simulink model "sgact"  (R2026b)
settings: Solver=FixedStepDiscrete  StopTime=inf  FixedStep=0.001
PreLoadFcn:
  | addpath(fullfile(fileparts(which('sgact')), 'matlab')); sgact_buses;
undefined symbols (not defined in the file or in its folder): sgact_sp_default
libraries: sgact_lib x4
settings Model: Creator=maccame  LastModifiedBy=maccame
settings SolverCC: ConcurrentTasks=on  PositivePriorityOrder=on
settings OptimizationCC: BlockReduction=off  DefaultParameterBehavior=Inlined  OptimizeBlockIOStorage=off
settings DebuggingCC: TasksWithSamePriorityMsg=none
settings HardwareCC: ProdHWDeviceType=Intel->x86-64 (Linux 64)  ProdLongLongMode=on
settings RTWCC: BuildConfiguration=Faster Runs  Description=Speedgoat Real-Time Target Machine  SystemTargetFile=speedgoat.tlc  TargetLang=C++  TemplateMakefile=slrealtime_default_tmf  Toolchain=Simulink Real-Time Toolchain
settings SimulinkRealTimeTargetCC: MATLABClassNameForMDSCustomization=Simulink.SoftwareTarget.GRTCustomization  TargetLangStandard=C++11 (ISO)

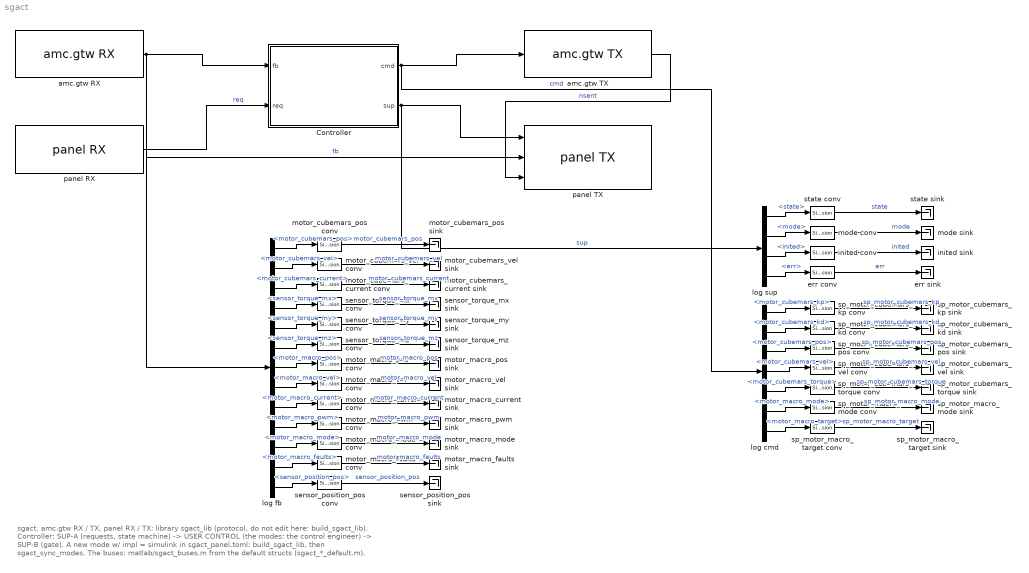
== system sgact ==
  note: sgact. amc.gtw RX / TX, panel RX / TX: library sgact_lib (protocol, do not edit here: build_sgact_lib).
      | Controller: SUP-A (requests, state machine) -> USER CONTROL (the modes: the control engineer) -> SUP-B (gate).
      | A new mode w/ impl = simulink in sgact_panel.toml: build_sgact_lib, then sgact_sync_modes.
      | The buses: matlab/sgact_buses.m from the default structs (sgact_*_default.m).
  Controller : Subsystem
  amc.gtw RX : sgact_lib/amc.gtw RX  SystemSampleTime=-1  VariantActivationTime=update diagram  EmptyChoice=off  PassThrough=off  PassThroughVariantControl=(default)  EmptyChoiceVariantControl=(default)  AllowFlexibleInterface=on  Latency=0  AutoFrameSizeCalculation=off
  amc.gtw TX : sgact_lib/amc.gtw TX  SystemSampleTime=-1  VariantActivationTime=update diagram  EmptyChoice=off  PassThrough=off  PassThroughVariantControl=(default)  EmptyChoiceVariantControl=(default)  AllowFlexibleInterface=on  Latency=0  AutoFrameSizeCalculation=off
  err conv : SignalConversion  OverrideOpt=off
  err sink : Terminator
  inited conv : SignalConversion  OverrideOpt=off
  inited sink : Terminator
  log cmd : BusSelector  OutputSignals=motor_cubemars_kp,motor_cubemars_kd,motor_cubemars_pos,motor_cubemars_vel,motor_cubemars_torque,motor_macro_mode,motor_macro_target
  log fb : BusSelector  OutputSignals=motor_cubemars_pos,motor_cubemars_vel,motor_cubemars_current,sensor_torque_mx,sensor_torque_my,sensor_torque_mz,motor_macro_pos,motor_macro_vel,motor_macro_current,motor_macro_pwm,motor_macro_mode,motor_macro_faults,sensor_position_pos
  log sup : BusSelector  OutputSignals=state,mode,inited,err
  mode conv : SignalConversion  OverrideOpt=off
  mode sink : Terminator
  motor_cubemars_current conv : SignalConversion  OverrideOpt=off
  motor_cubemars_current sink : Terminator
  motor_cubemars_pos conv : SignalConversion  OverrideOpt=off
  motor_cubemars_pos sink : Terminator
  motor_cubemars_vel conv : SignalConversion  OverrideOpt=off
  motor_cubemars_vel sink : Terminator
  motor_macro_current conv : SignalConversion  OverrideOpt=off
  motor_macro_current sink : Terminator
  motor_macro_faults conv : SignalConversion  OverrideOpt=off
  motor_macro_faults sink : Terminator
  motor_macro_mode conv : SignalConversion  OverrideOpt=off
  motor_macro_mode sink : Terminator
  motor_macro_pos conv : SignalConversion  OverrideOpt=off
  motor_macro_pos sink : Terminator
  motor_macro_pwm conv : SignalConversion  OverrideOpt=off
  motor_macro_pwm sink : Terminator
  motor_macro_vel conv : SignalConversion  OverrideOpt=off
  motor_macro_vel sink : Terminator
  panel RX : sgact_lib/panel RX  SystemSampleTime=-1  VariantActivationTime=update diagram  EmptyChoice=off  PassThrough=off  PassThroughVariantControl=(default)  EmptyChoiceVariantControl=(default)  AllowFlexibleInterface=on  Latency=0  AutoFrameSizeCalculation=off
  panel TX : sgact_lib/panel TX  SystemSampleTime=-1  VariantActivationTime=update diagram  EmptyChoice=off  PassThrough=off  PassThroughVariantControl=(default)  EmptyChoiceVariantControl=(default)  AllowFlexibleInterface=on  Latency=0  AutoFrameSizeCalculation=off
  sensor_position_pos conv : SignalConversion  OverrideOpt=off
  sensor_position_pos sink : Terminator
  sensor_torque_mx conv : SignalConversion  OverrideOpt=off
  sensor_torque_mx sink : Terminator
  sensor_torque_my conv : SignalConversion  OverrideOpt=off
  sensor_torque_my sink : Terminator
  sensor_torque_mz conv : SignalConversion  OverrideOpt=off
  sensor_torque_mz sink : Terminator
  sp_motor_cubemars_kd conv : SignalConversion  OverrideOpt=off
  sp_motor_cubemars_kd sink : Terminator
  sp_motor_cubemars_kp conv : SignalConversion  OverrideOpt=off
  sp_motor_cubemars_kp sink : Terminator
  sp_motor_cubemars_pos conv : SignalConversion  OverrideOpt=off
  sp_motor_cubemars_pos sink : Terminator
  sp_motor_cubemars_torque conv : SignalConversion  OverrideOpt=off
  sp_motor_cubemars_torque sink : Terminator
  sp_motor_cubemars_vel conv : SignalConversion  OverrideOpt=off
  sp_motor_cubemars_vel sink : Terminator
  sp_motor_macro_mode conv : SignalConversion  OverrideOpt=off
  sp_motor_macro_mode sink : Terminator
  sp_motor_macro_target conv : SignalConversion  OverrideOpt=off
  sp_motor_macro_target sink : Terminator
  state conv : SignalConversion  OverrideOpt=off
  state sink : Terminator
  wires:
  amc.gtw RX/1 -> Controller/1(fb), panel TX/2, log fb/1  "fb"
  panel RX/1 -> Controller/2(req)  "req"
  Controller/1(cmd) -> amc.gtw TX/1, log cmd/1  "cmd"
  Controller/2(sup) -> panel TX/1, log sup/1  "sup"
  amc.gtw TX/1 -> panel TX/3  "nsent"
  log sup/1 -> state conv/1  "<state>"
  state conv/1 -> state sink/1  "state"
  log sup/2 -> mode conv/1  "<mode>"
  mode conv/1 -> mode sink/1  "mode"
  log sup/3 -> inited conv/1  "<inited>"
  inited conv/1 -> inited sink/1  "inited"
  log sup/4 -> err conv/1  "<err>"
  err conv/1 -> err sink/1  "err"
  log cmd/1 -> sp_motor_cubemars_kp conv/1  "<motor_cubemars_kp>"
  sp_motor_cubemars_kp conv/1 -> sp_motor_cubemars_kp sink/1  "sp_motor_cubemars_kp"
  log cmd/2 -> sp_motor_cubemars_kd conv/1  "<motor_cubemars_kd>"
  sp_motor_cubemars_kd conv/1 -> sp_motor_cubemars_kd sink/1  "sp_motor_cubemars_kd"
  log cmd/3 -> sp_motor_cubemars_pos conv/1  "<motor_cubemars_pos>"
  sp_motor_cubemars_pos conv/1 -> sp_motor_cubemars_pos sink/1  "sp_motor_cubemars_pos"
  log cmd/4 -> sp_motor_cubemars_vel conv/1  "<motor_cubemars_vel>"
  sp_motor_cubemars_vel conv/1 -> sp_motor_cubemars_vel sink/1  "sp_motor_cubemars_vel"
  log cmd/5 -> sp_motor_cubemars_torque conv/1  "<motor_cubemars_torque>"
  sp_motor_cubemars_torque conv/1 -> sp_motor_cubemars_torque sink/1  "sp_motor_cubemars_torque"
  log cmd/6 -> sp_motor_macro_mode conv/1  "<motor_macro_mode>"
  sp_motor_macro_mode conv/1 -> sp_motor_macro_mode sink/1  "sp_motor_macro_mode"
  log cmd/7 -> sp_motor_macro_target conv/1  "<motor_macro_target>"
  sp_motor_macro_target conv/1 -> sp_motor_macro_target sink/1  "sp_motor_macro_target"
  log fb/1 -> motor_cubemars_pos conv/1  "<motor_cubemars_pos>"
  motor_cubemars_pos conv/1 -> motor_cubemars_pos sink/1  "motor_cubemars_pos"
  log fb/2 -> motor_cubemars_vel conv/1  "<motor_cubemars_vel>"
  motor_cubemars_vel conv/1 -> motor_cubemars_vel sink/1  "motor_cubemars_vel"
  log fb/3 -> motor_cubemars_current conv/1  "<motor_cubemars_current>"
  motor_cubemars_current conv/1 -> motor_cubemars_current sink/1  "motor_cubemars_current"
  log fb/4 -> sensor_torque_mx conv/1  "<sensor_torque_mx>"
  sensor_torque_mx conv/1 -> sensor_torque_mx sink/1  "sensor_torque_mx"
  log fb/5 -> sensor_torque_my conv/1  "<sensor_torque_my>"
  sensor_torque_my conv/1 -> sensor_torque_my sink/1  "sensor_torque_my"
  log fb/6 -> sensor_torque_mz conv/1  "<sensor_torque_mz>"
  sensor_torque_mz conv/1 -> sensor_torque_mz sink/1  "sensor_torque_mz"
  log fb/7 -> motor_macro_pos conv/1  "<motor_macro_pos>"
  motor_macro_pos conv/1 -> motor_macro_pos sink/1  "motor_macro_pos"
  log fb/8 -> motor_macro_vel conv/1  "<motor_macro_vel>"
  motor_macro_vel conv/1 -> motor_macro_vel sink/1  "motor_macro_vel"
  log fb/9 -> motor_macro_current conv/1  "<motor_macro_current>"
  motor_macro_current conv/1 -> motor_macro_current sink/1  "motor_macro_current"
  log fb/10 -> motor_macro_pwm conv/1  "<motor_macro_pwm>"
  motor_macro_pwm conv/1 -> motor_macro_pwm sink/1  "motor_macro_pwm"
  log fb/11 -> motor_macro_mode conv/1  "<motor_macro_mode>"
  motor_macro_mode conv/1 -> motor_macro_mode sink/1  "motor_macro_mode"
  log fb/12 -> motor_macro_faults conv/1  "<motor_macro_faults>"
  motor_macro_faults conv/1 -> motor_macro_faults sink/1  "motor_macro_faults"
  log fb/13 -> sensor_position_pos conv/1  "<sensor_position_pos>"
  sensor_position_pos conv/1 -> sensor_position_pos sink/1  "sensor_position_pos"

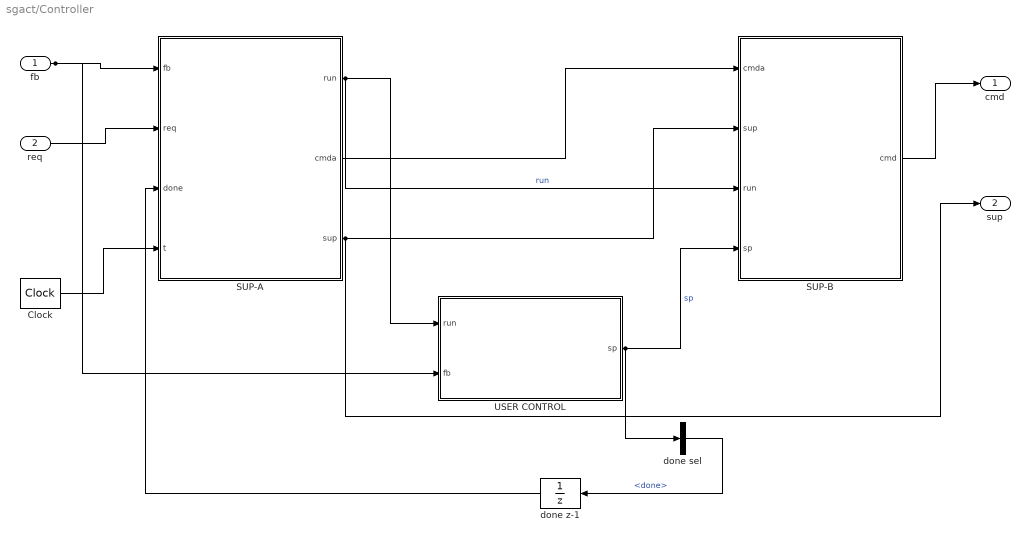
== system sgact/Controller ==
  fb : Inport  OutDataTypeStr=Bus: SGACT_FB  BusOutputAsStruct=on
  req : Inport  Port=2  OutDataTypeStr=Bus: SGACT_REQ  BusOutputAsStruct=on
  Clock : DigitalClock  SampleTime=0.001
  SUP-A : MATLAB Function  TreatAsAtomicUnit=on
  SUP-B : MATLAB Function  TreatAsAtomicUnit=on
  USER CONTROL : Subsystem
  done sel : BusSelector  OutputSignals=done
  done z-1 : UnitDelay  SampleTime=-1
  cmd : Outport
  sup : Outport  Port=2
  wires:
  fb/1 -> SUP-A/1(fb), USER CONTROL/2(fb)
  req/1 -> SUP-A/2(req)
  done z-1/1 -> SUP-A/3(done)
  Clock/1 -> SUP-A/4(t)
  SUP-A/1(run) -> USER CONTROL/1(run), SUP-B/3(run)  "run"
  SUP-A/2(cmda) -> SUP-B/1(cmda)
  SUP-A/3(sup) -> SUP-B/2(sup), sup/1
  USER CONTROL/1(sp) -> SUP-B/4(sp), done sel/1  "sp"
  done sel/1 -> done z-1/1  "<done>"
  SUP-B/1(cmd) -> cmd/1

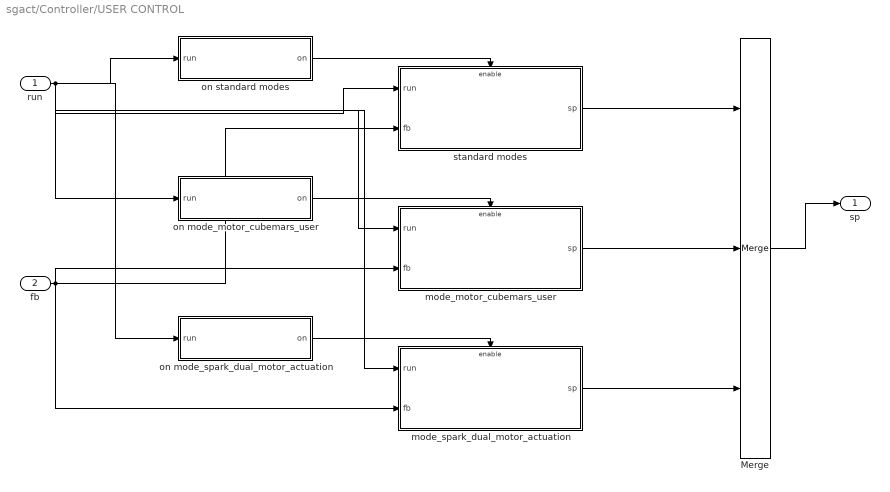
== system sgact/Controller/USER CONTROL ==
  run : Inport  OutDataTypeStr=Bus: SGACT_RUN  BusOutputAsStruct=on
  fb : Inport  Port=2  OutDataTypeStr=Bus: SGACT_FB  BusOutputAsStruct=on
  Merge : Merge  Inputs=3  InitialOutput=sgact_sp_default()
  mode_motor_cubemars_user : Subsystem
  mode_spark_dual_motor_actuation : Subsystem
  on mode_motor_cubemars_user : MATLAB Function  TreatAsAtomicUnit=on
  on mode_spark_dual_motor_actuation : MATLAB Function  TreatAsAtomicUnit=on
  on standard modes : MATLAB Function  TreatAsAtomicUnit=on
  standard modes : Subsystem
  sp : Outport
  wires:
  run/1 -> on standard modes/1(run), standard modes/1(run), on mode_motor_cubemars_user/1(run), mode_motor_cubemars_user/1(run), on mode_spark_dual_motor_actuation/1(run), mode_spark_dual_motor_actuation/1(run)
  on standard modes/1(on) -> standard modes/Enable
  fb/1 -> standard modes/2(fb), mode_motor_cubemars_user/2(fb), mode_spark_dual_motor_actuation/2(fb)
  on mode_motor_cubemars_user/1(on) -> mode_motor_cubemars_user/Enable
  on mode_spark_dual_motor_actuation/1(on) -> mode_spark_dual_motor_actuation/Enable
  standard modes/1(sp) -> Merge/1
  mode_motor_cubemars_user/1(sp) -> Merge/2
  mode_spark_dual_motor_actuation/1(sp) -> Merge/3
  Merge/1 -> sp/1

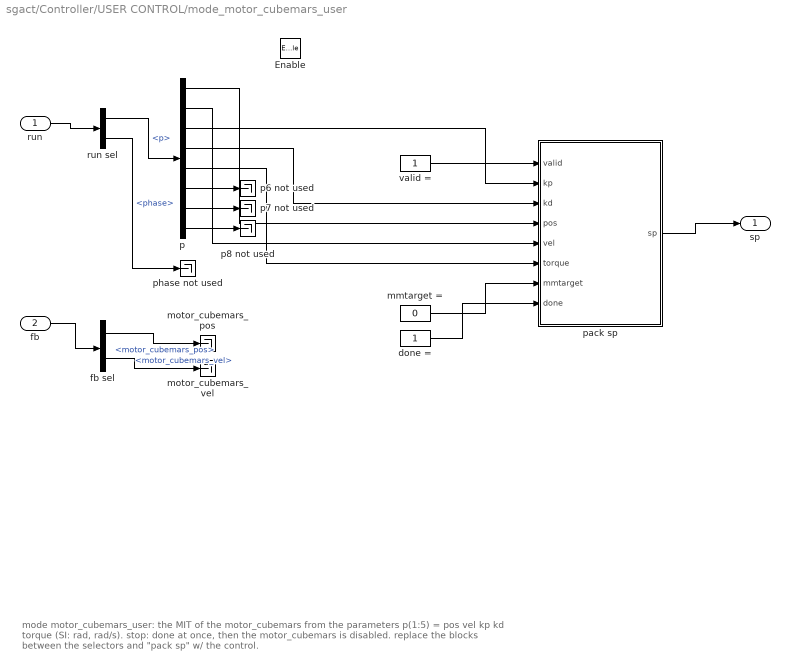
== system sgact/Controller/USER CONTROL/mode_motor_cubemars_user ==
  note: mode motor_cubemars_user: the MIT of the motor_cubemars from the parameters
      | p(1:5) = pos vel kp kd torque (SI: rad, rad/s). stop: done at once, then the motor_cubemars is disabled.
      | replace the blocks between the selectors and "pack sp" w/ the control.
  run : Inport  OutDataTypeStr=Bus: SGACT_RUN  BusOutputAsStruct=on
  fb : Inport  Port=2  OutDataTypeStr=Bus: SGACT_FB  BusOutputAsStruct=on
  Enable : EnablePort  StatesWhenEnabling=reset
  done = : Constant
  fb sel : BusSelector  OutputSignals=motor_cubemars_pos,motor_cubemars_vel
  mmtarget = : Constant  Value=0
  motor_cubemars_pos : Terminator
  motor_cubemars_vel : Terminator
  p : Demux  Outputs=8
  p6 not used : Terminator
  p7 not used : Terminator
  p8 not used : Terminator
  pack sp : MATLAB Function  TreatAsAtomicUnit=on
  phase not used : Terminator
  run sel : BusSelector  OutputSignals=p,phase
  valid = : Constant
  sp : Outport  OutDataTypeStr=Bus: SGACT_SP  InitialOutput=sgact_sp_default()
  wires:
  run/1 -> run sel/1
  run sel/1 -> p/1  "<p>"
  run sel/2 -> phase not used/1  "<phase>"
  fb/1 -> fb sel/1
  fb sel/1 -> motor_cubemars_pos/1  "<motor_cubemars_pos>"
  fb sel/2 -> motor_cubemars_vel/1  "<motor_cubemars_vel>"
  pack sp/1(sp) -> sp/1
  valid =/1 -> pack sp/1(valid)
  p/3 -> pack sp/2(kp)
  p/4 -> pack sp/3(kd)
  p/1 -> pack sp/4(pos)
  p/2 -> pack sp/5(vel)
  p/5 -> pack sp/6(torque)
  mmtarget =/1 -> pack sp/7(mmtarget)
  done =/1 -> pack sp/8(done)
  p/6 -> p6 not used/1
  p/7 -> p7 not used/1
  p/8 -> p8 not used/1

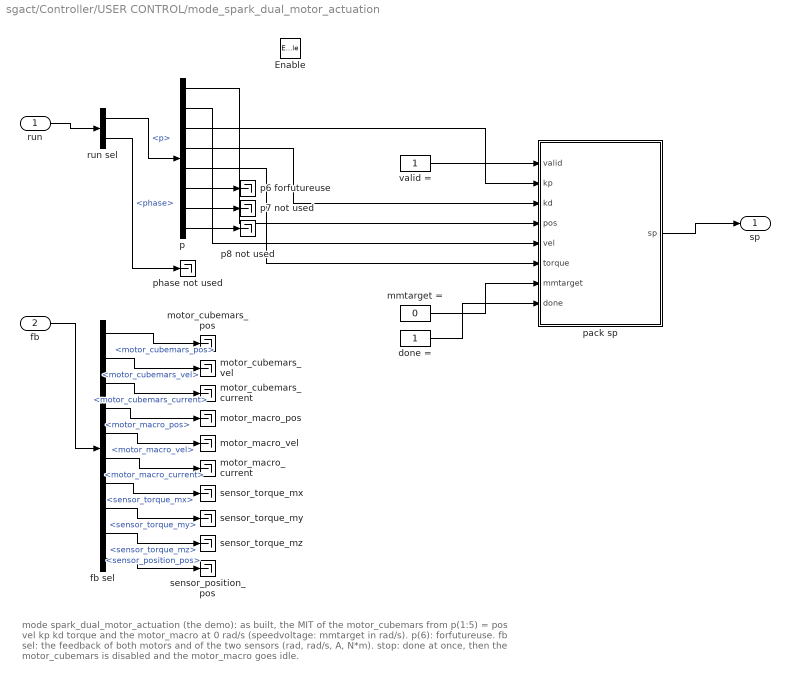
== system sgact/Controller/USER CONTROL/mode_spark_dual_motor_actuation ==
  note: mode spark_dual_motor_actuation (the demo): as built, the MIT of the motor_cubemars from p(1:5) = pos vel kp kd torque
      | and the motor_macro at 0 rad/s (speedvoltage: mmtarget in rad/s). p(6): forfutureuse.
      | fb sel: the feedback of both motors and of the two sensors (rad, rad/s, A, N*m).
      | stop: done at once, then the motor_cubemars is disabled and the motor_macro goes idle.
  run : Inport  OutDataTypeStr=Bus: SGACT_RUN  BusOutputAsStruct=on
  fb : Inport  Port=2  OutDataTypeStr=Bus: SGACT_FB  BusOutputAsStruct=on
  Enable : EnablePort  StatesWhenEnabling=reset
  done = : Constant
  fb sel : BusSelector  OutputSignals=motor_cubemars_pos,motor_cubemars_vel,motor_cubemars_current,motor_macro_pos,motor_macro_vel,motor_macro_current,sensor_torque_mx,sensor_torque_my,sensor_torque_mz,sensor_position_pos
  mmtarget = : Constant  Value=0
  motor_cubemars_current : Terminator
  motor_cubemars_pos : Terminator
  motor_cubemars_vel : Terminator
  motor_macro_current : Terminator
  motor_macro_pos : Terminator
  motor_macro_vel : Terminator
  p : Demux  Outputs=8
  p6 forfutureuse : Terminator
  p7 not used : Terminator
  p8 not used : Terminator
  pack sp : MATLAB Function  TreatAsAtomicUnit=on
  phase not used : Terminator
  run sel : BusSelector  OutputSignals=p,phase
  sensor_position_pos : Terminator
  sensor_torque_mx : Terminator
  sensor_torque_my : Terminator
  sensor_torque_mz : Terminator
  valid = : Constant
  sp : Outport  OutDataTypeStr=Bus: SGACT_SP  InitialOutput=sgact_sp_default()
  wires:
  run/1 -> run sel/1
  run sel/1 -> p/1  "<p>"
  run sel/2 -> phase not used/1  "<phase>"
  fb/1 -> fb sel/1
  fb sel/1 -> motor_cubemars_pos/1  "<motor_cubemars_pos>"
  fb sel/2 -> motor_cubemars_vel/1  "<motor_cubemars_vel>"
  fb sel/3 -> motor_cubemars_current/1  "<motor_cubemars_current>"
  fb sel/4 -> motor_macro_pos/1  "<motor_macro_pos>"
  fb sel/5 -> motor_macro_vel/1  "<motor_macro_vel>"
  fb sel/6 -> motor_macro_current/1  "<motor_macro_current>"
  fb sel/7 -> sensor_torque_mx/1  "<sensor_torque_mx>"
  fb sel/8 -> sensor_torque_my/1  "<sensor_torque_my>"
  fb sel/9 -> sensor_torque_mz/1  "<sensor_torque_mz>"
  fb sel/10 -> sensor_position_pos/1  "<sensor_position_pos>"
  pack sp/1(sp) -> sp/1
  valid =/1 -> pack sp/1(valid)
  p/3 -> pack sp/2(kp)
  p/4 -> pack sp/3(kd)
  p/1 -> pack sp/4(pos)
  p/2 -> pack sp/5(vel)
  p/5 -> pack sp/6(torque)
  mmtarget =/1 -> pack sp/7(mmtarget)
  done =/1 -> pack sp/8(done)
  p/6 -> p6 forfutureuse/1
  p/7 -> p7 not used/1
  p/8 -> p8 not used/1

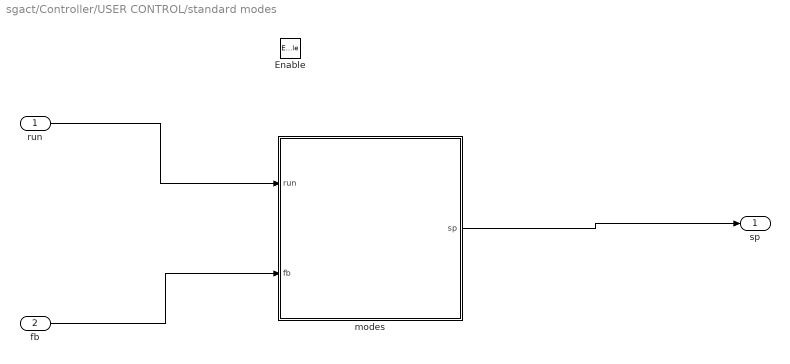
== system sgact/Controller/USER CONTROL/standard modes ==
  run : Inport  OutDataTypeStr=Bus: SGACT_RUN  BusOutputAsStruct=on
  fb : Inport  Port=2  OutDataTypeStr=Bus: SGACT_FB  BusOutputAsStruct=on
  Enable : EnablePort  StatesWhenEnabling=reset
  modes : MATLAB Function  TreatAsAtomicUnit=on
  sp : Outport  OutDataTypeStr=Bus: SGACT_SP  InitialOutput=sgact_sp_default()
  wires:
  run/1 -> modes/1(run)
  fb/1 -> modes/2(fb)
  modes/1(sp) -> sp/1

== matlab function sgact/Controller/SUP-B ==
  data: cmda input Bus: SGACT_CMD; cmd output Bus: SGACT_CMD; sup input Bus: SGACT_SUP; run input Bus: SGACT_RUN; sp input Bus: SGACT_SP
function cmd = supb(cmda, sup, run, sp)
%#codegen
% the gate: which setpoints of the mode leave. see matlab/sgact_sup_b.m
cmd = sgact_sup_b(cmda, sup, run, sp);

== matlab function sgact/Controller/SUP-A ==
  data: fb input Bus: SGACT_FB; run output Bus: SGACT_RUN; req input Bus: SGACT_REQ; done input; t input; cmda output Bus: SGACT_CMD; sup output Bus: SGACT_SUP
function [run, cmda, sup] = supa(fb, req, done, t)
%#codegen
% the requests, the watchdogs, the state machine, the rpc: see matlab/sgact_sup_a.m
[run, cmda, sup] = sgact_sup_a(fb, req, done, t);

== matlab function sgact/Controller/USER CONTROL/standard modes/modes ==
  data: run input Bus: SGACT_RUN; sp output Bus: SGACT_SP; fb input Bus: SGACT_FB
function sp = modes(run, fb)
%#codegen
% the modes w/ impl = matlab of sgact_panel.toml: matlab/sgact_mode_<name>.m
sp = sgact_std_modes(run, fb);

== matlab function sgact/Controller/USER CONTROL/mode_motor_cubemars_user/pack sp ==
  data: valid input; sp output Bus: SGACT_SP; kp input; kd input; pos input; vel input; torque input; mmtarget input; done input
function sp = pack(valid, kp, kd, pos, vel, torque, mmtarget, done)
%#codegen
% the bus SGACT_SP from 8 scalars. valid: a MIT for the motor_cubemars (kp kd pos vel torque, SI);
% mmtarget: the setpoint of the motor_macro (modes w/ a controlmode); done: (stop) the exit is over
sp = sgact_sp_default();
sp.valid = valid ~= 0;
sp.kp = double(kp); sp.kd = double(kd); sp.pos = double(pos); sp.vel = double(vel); sp.torque = double(torque);
sp.mmtarget = double(mmtarget);
sp.done = done ~= 0;

== matlab function sgact/Controller/USER CONTROL/mode_spark_dual_motor_actuation/pack sp ==
  data: valid input; sp output Bus: SGACT_SP; kp input; kd input; pos input; vel input; torque input; mmtarget input; done input
function sp = pack(valid, kp, kd, pos, vel, torque, mmtarget, done)
%#codegen
% the bus SGACT_SP from 8 scalars. valid: a MIT for the motor_cubemars (kp kd pos vel torque, SI);
% mmtarget: the setpoint of the motor_macro (modes w/ a controlmode); done: (stop) the exit is over
sp = sgact_sp_default();
sp.valid = valid ~= 0;
sp.kp = double(kp); sp.kd = double(kd); sp.pos = double(pos); sp.vel = double(vel); sp.torque = double(torque);
sp.mmtarget = double(mmtarget);
sp.done = done ~= 0;

== matlab function sgact/Controller/USER CONTROL/on standard modes ==
  data: run input Bus: SGACT_RUN; on output
function on = f(run)
%#codegen
% the block "standard modes" runs while a mode w/ impl = matlab runs or stops
on = sgact_std_on(run);

== matlab function sgact/Controller/USER CONTROL/on mode_motor_cubemars_user ==
  data: run input Bus: SGACT_RUN; on output
function on = f(run)
%#codegen
% mode_motor_cubemars_user (id 3 of sgact_panel.toml) runs while that mode runs or stops
on = run.phase > 0 && run.mode == 3;

== matlab function sgact/Controller/USER CONTROL/on mode_spark_dual_motor_actuation ==
  data: run input Bus: SGACT_RUN; on output
function on = f(run)
%#codegen
% mode_spark_dual_motor_actuation (id 20 of sgact_panel.toml) runs while that mode runs or stops
on = run.phase > 0 && run.mode == 20;
